simulink model "kalman_simple"  (R2025b)
settings: Solver=FixedStepDiscrete  StartTime=0.0  StopTime=30  FixedStep=0.1  RelTol=1e-3
settings Model: Creator=alosw  LastModifiedBy=alosw

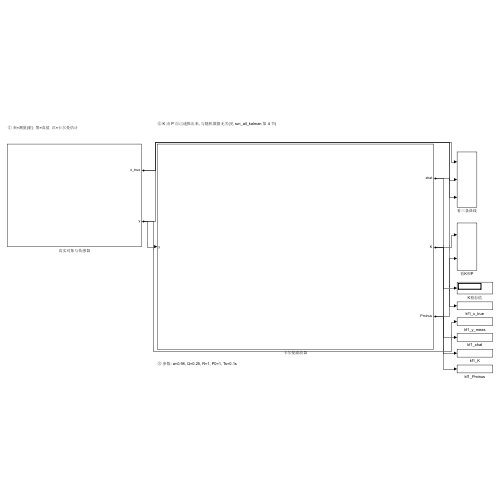
[thumbnail: Simulink's stored preview of the top-level diagram]
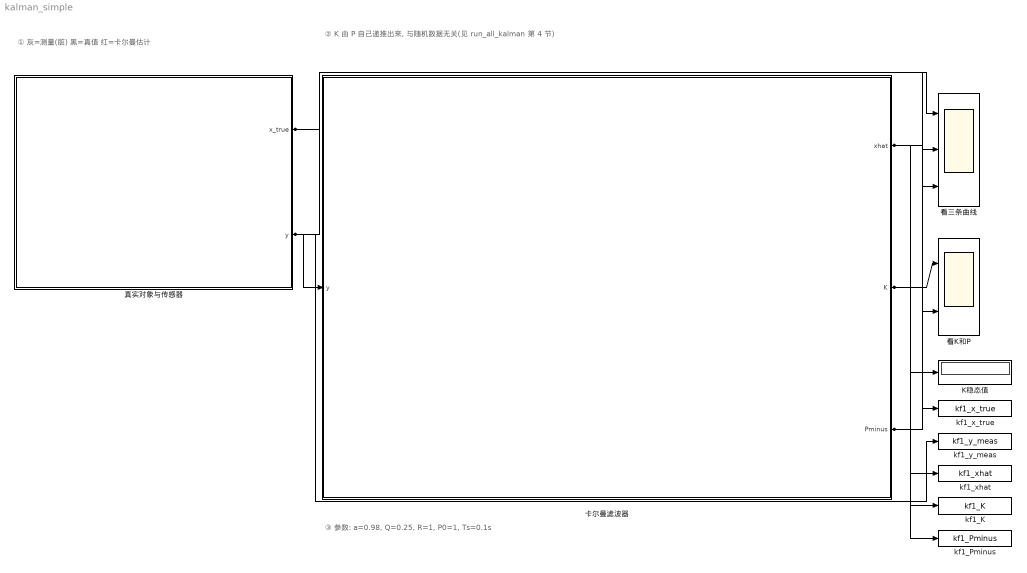
== system kalman_simple ==
  note: ① 灰=测量(脏) 黑=真值 红=卡尔曼估计
  note: ② K 由 P 自己递推出来, 与随机数据无关(见 run_all_kalman 第 4 节)
  note: ③ 参数: a=0.98, Q=0.25, R=1, P0=1, Ts=0.1s
  K稳态值 : Display
  kf1_K : ToWorkspace  VariableName=kf1_K  SaveFormat=Timeseries  SampleTime=-1
  kf1_Pminus : ToWorkspace  VariableName=kf1_Pminus  SaveFormat=Timeseries  SampleTime=-1
  kf1_x_true : ToWorkspace  VariableName=kf1_x_true  SaveFormat=Timeseries  SampleTime=-1
  kf1_xhat : ToWorkspace  VariableName=kf1_xhat  SaveFormat=Timeseries  SampleTime=-1
  kf1_y_meas : ToWorkspace  VariableName=kf1_y_meas  SaveFormat=Timeseries  SampleTime=-1
  卡尔曼滤波器 : Subsystem
  看K和P : Scope  NumInputPorts=2
  看三条曲线 : Scope  NumInputPorts=3
  真实对象与传感器 : Subsystem
  wires:
  真实对象与传感器/1(x_true) -> 看三条曲线/1, kf1_x_true/1
  真实对象与传感器/2(y) -> 看三条曲线/2, kf1_y_meas/1, 卡尔曼滤波器/1(y)
  卡尔曼滤波器/1(xhat) -> 看三条曲线/3, kf1_xhat/1
  卡尔曼滤波器/2(K) -> 看K和P/1, K稳态值/1, kf1_K/1
  卡尔曼滤波器/3(Pminus) -> 看K和P/2, kf1_Pminus/1

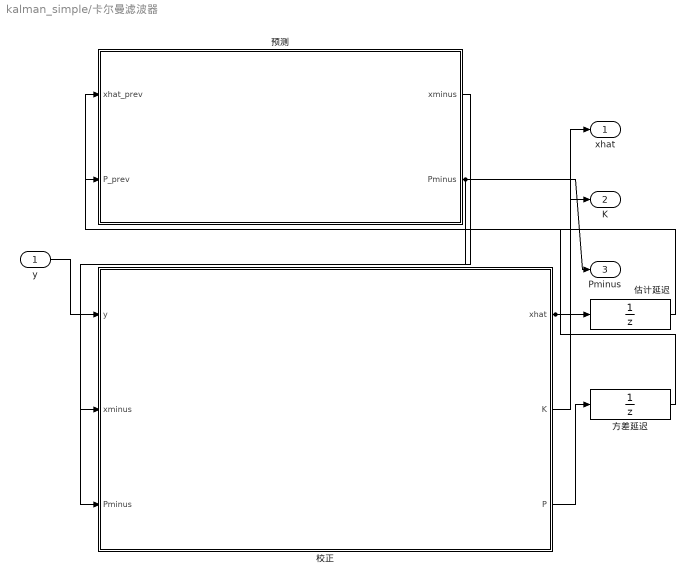
== system kalman_simple/卡尔曼滤波器 ==
  y : Inport
  估计延迟 : UnitDelay  SampleTime=0.1  HasFrameUpgradeWarning=on
  方差延迟 : UnitDelay  InitialCondition=1  SampleTime=0.1  HasFrameUpgradeWarning=on
  校正 : Subsystem
  预测 : Subsystem
  xhat : Outport
  K : Outport  Port=2
  Pminus : Outport  Port=3
  wires:
  估计延迟/1 -> 预测/1(xhat_prev)
  方差延迟/1 -> 预测/2(P_prev)
  y/1 -> 校正/1(y)
  预测/1(xminus) -> 校正/2(xminus)
  预测/2(Pminus) -> 校正/3(Pminus), Pminus/1
  校正/1(xhat) -> xhat/1, 估计延迟/1
  校正/2(K) -> K/1
  校正/3(P) -> 方差延迟/1

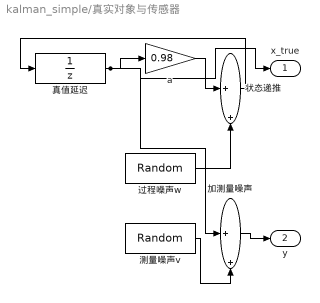
== system kalman_simple/真实对象与传感器 ==
  a : Gain  Gain=0.98
  加测量噪声 : Sum  Inputs=|++
  测量噪声v : RandomNumber  Seed=9871  SampleTime=0.1
  状态递推 : Sum  Inputs=|++
  真值延迟 : UnitDelay  InitialCondition=1  SampleTime=0.1  HasFrameUpgradeWarning=on
  过程噪声w : RandomNumber  Variance=0.25  Seed=23341  SampleTime=0.1
  x_true : Outport
  y : Outport  Port=2
  wires:
  真值延迟/1 -> a/1, 加测量噪声/1, x_true/1
  a/1 -> 状态递推/1
  过程噪声w/1 -> 状态递推/2
  状态递推/1 -> 真值延迟/1
  测量噪声v/1 -> 加测量噪声/2
  加测量噪声/1 -> y/1

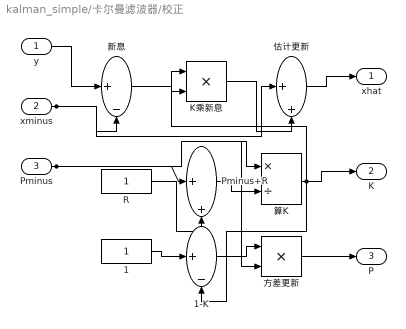
== system kalman_simple/卡尔曼滤波器/校正 ==
  y : Inport
  xminus : Inport  Port=2
  Pminus : Inport  Port=3
  1 : Constant
  1-K : Sum  Inputs=|+-
  K乘新息 : Product  Inputs=**
  Pminus+R : Sum  Inputs=|++
  R : Constant
  估计更新 : Sum  Inputs=|++
  新息 : Sum  Inputs=|+-
  方差更新 : Product  Inputs=**
  算K : Product  Inputs=*/
  xhat : Outport
  K : Outport  Port=2
  P : Outport  Port=3
  wires:
  y/1 -> 新息/1
  xminus/1 -> 新息/2, 估计更新/1
  Pminus/1 -> Pminus+R/1, 算K/1, 方差更新/2
  R/1 -> Pminus+R/2
  Pminus+R/1 -> 算K/2
  算K/1 -> K/1, K乘新息/1, 1-K/2
  新息/1 -> K乘新息/2
  K乘新息/1 -> 估计更新/2
  估计更新/1 -> xhat/1
  1/1 -> 1-K/1
  1-K/1 -> 方差更新/1
  方差更新/1 -> P/1

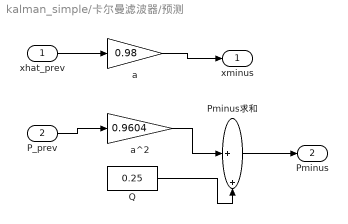
== system kalman_simple/卡尔曼滤波器/预测 ==
  xhat_prev : Inport
  P_prev : Inport  Port=2
  Pminus求和 : Sum  Inputs=|++
  Q : Constant  Value=0.25
  a : Gain  Gain=0.98
  a^2 : Gain  Gain=0.9604
  xminus : Outport
  Pminus : Outport  Port=2
  wires:
  xhat_prev/1 -> a/1
  a/1 -> xminus/1
  P_prev/1 -> a^2/1
  a^2/1 -> Pminus求和/1
  Q/1 -> Pminus求和/2
  Pminus求和/1 -> Pminus/1
